simulink library "Steer_Rack"  (R2025a)
settings: Solver=VariableStepAuto  StartTime=0.0  StopTime=10.0  RelTol=1e-3
undefined symbols (not defined in the file): Vehicle
libraries: Steer_Rack_None x1, Steer_Rack_Only x1, Steer_Rack_RackDrivenShafts x1, Steer_Rack_RackStaticShafts x1, Steer_Rack_Wheel x1, Steer_Rack_WheelByWire x1, Steer_Rack_Wheel_Indep x1, Steer_Rack_WheelVarRatio x1, Steer_Rack_WheelDrivenRack x1, Steer_Rack_WheelDrivenRack1UJoint x1, Vehicle_Inputs x1
Description:
  | Component of Simscape Vehicle Templates Library
  | 
  | Copyright 2018-2026 The MathWorks, Inc.
settings Model: Creator=smiller  LastModifiedBy=smiller
settings SolverCC: AlgebraicLoopSolver=TrustRegion
settings DataIOCC: ReturnWorkspaceOutputs=off
settings OptimizationCC: ReuseModelBlockBuffer=off
settings DebuggingCC: UnconnectedInputMsg=warning  UnconnectedOutputMsg=warning  UnconnectedLineMsg=warning  ArithmeticOperatorsInVariantConditions=warning
settings ModelReferenceCC: EnableRefExpFcnMdlSchedulingChecks=on
settings SFSimCC: CustomCodeUndefinedFunction=UseInterfaceOnly
settings RTWCC: GPUComputeCapability=3.5  DLArmComputeVersion=19.05

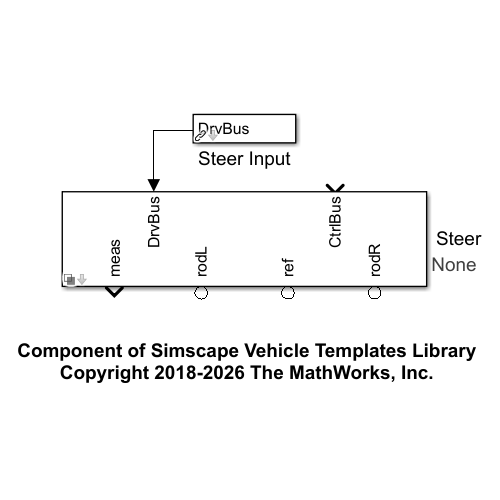
[thumbnail: Simulink's stored preview of the top-level diagram]
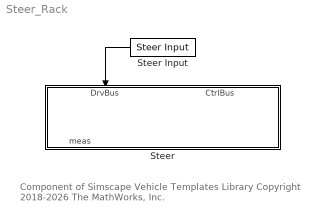
== system Steer_Rack ==
  note: Component of Simscape Vehicle Templates Library
      | Copyright 2018-2026 The MathWorks, Inc.
  Steer : Subsystem  Variant=on  VariantControlMode=label  VariantControl=Steer  LabelModeActiveChoice=None  mask(Steering System with Rack){Steer=Vehicle.Chassis.SuspF.Steer, VariantLabel=Vehicle.Chassis.SuspF.Steer.class.Value}
      mask prompts: Steer "Steer Parameters"; VariantLabel "Variant Label"
      mask help: Models steering system that involves a rack. Optionally include steering wheel. Connection between steering wheel and rack can be mechanical, specified by a lookup table, or a control system as in steer-by-wire. Option is chosen by string provided in Variant Label. The parameters for the selected option are contained in Steer data structure.
      mask init:
      | curblk = gcb;
      | 
      | % Set variant for this block 
      | set_param(curblk,'LabelModeActiveChoice',VariantLabel);
      settings: AttributesFormatString=%<ActiveVariant>
      mask Display: disp(' ');
  Steer Input : Vehicle_Inputs/DrvBus/Steer Input  popup_steer_input=Sequence
  wires:
  Steer Input/1 -> Steer/1(DrvBus)

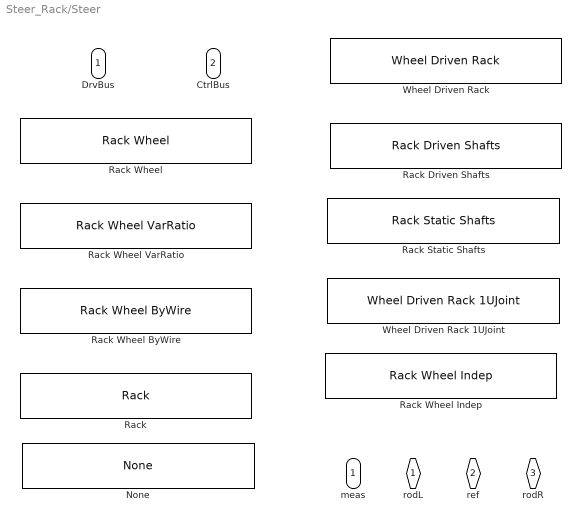
== system Steer_Rack/Steer ==
  DrvBus : Inport
  CtrlBus : Inport  Port=2
  None : Steer_Rack_None/None  SystemSampleTime=-1  VariantControl=None  VariantActivationTime=update diagram  EmptyChoice=off  PassThrough=off  PassThroughVariantControl=(default)  EmptyChoiceVariantControl=(default)  AllowFlexibleInterface=on  Latency=0  AutoFrameSizeCalculation=off
  Rack : Steer_Rack_Only/Rack  Tag=PublishSubsystem  VariantControl=Rack  hp_mt_rack=Steer.Rack.sMount.Value  hp_out_rack=Steer.Rack.sOutboard.Value  rack_mass=Steer.Rack.m.Value  whl2rack_whlangle=Steer.Ratio_Table.aWheel.Value  whl2rack_rackdisp=Steer.Ratio_Table.xRack.Value  whl2rack_filter=1/Steer.Rack.fActuatorCutoff.Value  clr_rack=Visual.SteeringRack.clr  opc_rack=Visual.part.opc  radius_rack=Visual.SteeringRack.rad  clr_connhp=Visual.hp.clr  opc_connhp=Visual.hp.opc  size_connhp=Visual.hp.rad
  Rack Driven Shafts : Steer_Rack_RackDrivenShafts/Rack Driven Shafts  Tag=PublishSubsystem  VariantControl=RackDrivenShafts  hp_wheel=Steer.Wheel.sMount.Value  wheel_axis_incl=Steer.Wheel.aAxis.Value  hp_mt_rack=Steer.Rack.sMount.Value  hp_out_rack=Steer.Rack.sOutboard.Value  hp_pinion=Steer.Pinion.sMount.Value  Wheel=Steer.Wheel  len_sha_u=Steer.Shaft_Upper.xLength.Value  sha_u_mass=Steer.Shaft_Upper.m.Value  sha_i_mass=Steer.Shaft_Intermediate.m.Value  len_sha_l=Steer.Shaft_Lower.xLength.Value  sha_l_mass=Steer.Shaft_Lower.m.Value  rad_pinion=Steer.Pinion.xRad.Value  pinion_mass=Steer.Pinion.m.Value  rack_mass=Steer.Rack.m.Value  whl2rack_whlangle=Steer.Ratio_Table.aWheel.Value  whl2rack_rackdisp=Steer.Ratio_Table.xRack.Value  steer_filter=1/Steer.Rack.fActuatorCutoff.Value  clr_rack=Visual.SteeringRack.clr  opc_rack=Visual.part.opc  radius_rack=Visual.SteeringRack.rad  clr_shaft=Visual.SteeringShafts.clr  opc_shaft=Visual.part.opc  size_shaft=Visual.SteeringShafts.rad  clr_pinion=Visual.SteeringPinion.clr  opc_pinion=Visual.part.opc  len_pinion=Visual.SteeringPinion.len  clr_connhp=Visual.hp.clr  opc_connhp=Visual.hp.opc  size_connhp=Visual.hp.rad  clr_wheel=Visual.SteeringWheel.clr  opc_wheel=Visual.part.opc  DriverHuman=Steer.DriverHuman
  Rack Static Shafts : Steer_Rack_RackStaticShafts/Rack Static Shafts  Tag=PublishSubsystem  VariantControl=RackStaticShafts  hp_wheel=Steer.Wheel.sMount.Value  wheel_axis_incl=Steer.Wheel.aAxis.Value  hp_mt_rack=Steer.Rack.sMount.Value  hp_out_rack=Steer.Rack.sOutboard.Value  hp_pinion=Steer.Pinion.sMount.Value  Wheel=Steer.Wheel  len_sha_u=Steer.Shaft_Upper.xLength.Value  sha_u_mass=Steer.Shaft_Upper.m.Value  sha_i_mass=Steer.Shaft_Intermediate.m.Value  len_sha_l=Steer.Shaft_Lower.xLength.Value  sha_l_mass=Steer.Shaft_Lower.m.Value  rad_pinion=Steer.Pinion.xRad.Value  pinion_mass=Steer.Pinion.m.Value  rack_mass=Steer.Rack.m.Value  whl2rack_whlangle=Steer.Ratio_Table.aWheel.Value  whl2rack_rackdisp=Steer.Ratio_Table.xRack.Value  steer_filter=1/Steer.Rack.fActuatorCutoff.Value  clr_rack=Visual.SteeringRack.clr  opc_rack=Visual.part.opc  radius_rack=Visual.SteeringRack.rad  clr_solid=Visual.SteeringShafts.clr  opc_solid=Visual.part.opc  rad_solid=Visual.SteeringShafts.rad  clr_pinion=Visual.SteeringPinion.clr  opc_pinion=Visual.part.opc  len_pinion=Visual.SteeringPinion.len  clr_connhp=Visual.hp.clr  opc_connhp=Visual.hp.opc  size_connhp=Visual.hp.rad  clr_wheel=Visual.SteeringWheel.clr  opc_wheel=Visual.part.opc  DriverHuman=Steer.DriverHuman
  Rack Wheel : Steer_Rack_Wheel/Rack Wheel  Tag=PublishSubsystem  VariantControl=RackWheel  hp_wheel=Steer.Wheel.sMount.Value  wheel_axis_incl=Steer.Wheel.aAxis.Value  hp_mt_rack=Steer.Rack.sMount.Value  hp_out_rack=Steer.Rack.sOutboard.Value  Wheel=Steer.Wheel  rack_mass=Steer.Rack.m.Value  whl2rack_whlangle=Steer.Ratio_Table.aWheel.Value  whl2rack_rackdisp=Steer.Ratio_Table.xRack.Value  whl2rack_filter=1/Steer.Rack.fActuatorCutoff.Value  clr_rack=Visual.SteeringRack.clr  opc_rack=Visual.part.opc  radius_rack=Visual.SteeringRack.rad  clr_connhp=Visual.hp.clr  opc_connhp=Visual.hp.opc  size_connhp=Visual.hp.rad  clr_wheel=Visual.SteeringWheel.clr  opc_wheel=Visual.part.opc  DriverHuman=Steer.DriverHuman
  Rack Wheel ByWire : Steer_Rack_WheelByWire/Rack Wheel ByWire  Tag=PublishSubsystem  VariantControl=RackWheelByWire  hp_wheel=Steer.Wheel.sMount.Value  wheel_axis_incl=Steer.Wheel.aAxis.Value  hp_mt_rack=Steer.Rack.sMount.Value  hp_out_rack=Steer.Rack.sOutboard.Value  Wheel=Steer.Wheel  rack_mass=Steer.Rack.m.Value  whl2rack_filter=1/Steer.Rack.fActuatorCutoff.Value  clr_rack=Visual.SteeringRack.clr  opc_rack=Visual.part.opc  radius_rack=Visual.SteeringRack.rad  clr_connhp=Visual.hp.clr  opc_connhp=Visual.hp.opc  size_connhp=Visual.hp.rad  clr_wheel=Visual.SteeringWheel.clr  opc_wheel=Visual.part.opc  DriverHuman=Steer.DriverHuman  Kp_breakpoints=Steer.Control.KpTable.xRack.Value  Kp_values=Steer.Control.KpTable.Kp.Value  Ki=Steer.Control.Ki.Value  Kd=Steer.Control.Kd.Value  tFilt_xRack=1/Steer.Control.fRackxCutoff.Value  tFilt_deriv=1/Steer.Control.fErrDerCutoff.Value  nTrqSteer=Steer.Control.nSteerTrq.Value  vDC=Steer.vMotor.Value  mSteer_trq=Steer.MotorSteer.TorqueSpd.trq.Value  mSteer_spd=Steer.MotorSteer.TorqueSpd.w.Value  mSteer_tc=1/Steer.MotorSteer.fActuatorCutoff.Value  mSteer_J=Steer.MotorSteer.J.Value  mSteer_d=Steer.MotorSteer.D.Value  mRack_trq=Steer.MotorRack.TorqueSpd.trq.Value  mRack_spd=Steer.MotorRack.TorqueSpd.w.Value  mRack_tc=1/Steer.MotorRack.fActuatorCutoff.Value  mRack_J=Steer.MotorRack.J.Value  mRack_d=Steer.MotorRack.D.Value  kRackCompliance=Steer.Rack.kCompliance.Value  DRackCompliance=Steer.Rack.DCompliance.Value  rPinion=Steer.Rack.xPinionRadius.Value  DRack=Steer.Rack.DHousing.Value
  Rack Wheel Indep : Steer_Rack_Wheel_Indep/Rack Wheel Indep  Tag=PublishSubsystem  VariantControl=RackWheelIndep  hp_wheel=Steer.Wheel.sMount.Value  wheel_axis_incl=Steer.Wheel.aAxis.Value  hp_mt_rack=Steer.Rack.sMount.Value  hp_out_rack=Steer.Rack.sOutboard.Value  Wheel=Steer.Wheel  rack_mass=Steer.Rack.m.Value  whl2rack_filter=1/Steer.Rack.fActuatorCutoff.Value  clr_rack=Visual.SteeringRack.clr  opc_rack=Visual.part.opc  radius_rack=Visual.SteeringRack.rad  clr_connhp=Visual.hp.clr  opc_connhp=Visual.hp.opc  size_connhp=Visual.hp.rad  clr_wheel=Visual.SteeringWheel.clr  opc_wheel=Visual.part.opc  DriverHuman=Steer.DriverHuman
  Rack Wheel VarRatio : Steer_Rack_WheelVarRatio/Rack Wheel VarRatio  Tag=PublishSubsystem  VariantControl=RackWheelVarRatio  hp_wheel=Steer.Wheel.sMount.Value  wheel_axis_incl=Steer.Wheel.aAxis.Value  hp_mt_rack=Steer.Rack.sMount.Value  hp_out_rack=Steer.Rack.sOutboard.Value  Wheel=Steer.Wheel  rack_mass=Steer.Rack.m.Value  whl2rack_filter=1/Steer.Rack.fActuatorCutoff.Value  clr_rack=Visual.SteeringRack.clr  opc_rack=Visual.part.opc  radius_rack=Visual.SteeringRack.rad  clr_connhp=Visual.hp.clr  opc_connhp=Visual.hp.opc  size_connhp=Visual.hp.rad  clr_wheel=Visual.SteeringWheel.clr  opc_wheel=Visual.part.opc  DriverHuman=Steer.DriverHuman  nTrqSteer=Steer.Control.nSteerTrq.Value  tFilt_forceFeedback=1/Steer.Control.fForceCutoff.Value
  Wheel Driven Rack : Steer_Rack_WheelDrivenRack/Wheel Driven Rack  Tag=PublishSubsystem  VariantControl=WheelDrivenRack  hp_wheel=Steer.Wheel.sMount.Value  wheel_axis_incl=Steer.Wheel.aAxis.Value  hp_mt_rack=Steer.Rack.sMount.Value  hp_out_rack=Steer.Rack.sOutboard.Value  hp_pinion=Steer.Pinion.sMount.Value  Wheel=Steer.Wheel  len_sha_u=Steer.Shaft_Upper.xLength.Value  sha_u_mass=Steer.Shaft_Upper.m.Value  sha_i_mass=Steer.Shaft_Intermediate.m.Value  len_sha_l=Steer.Shaft_Lower.xLength.Value  sha_l_mass=Steer.Shaft_Lower.m.Value  rad_pinion=Steer.Pinion.xRad.Value  pinion_mass=Steer.Pinion.m.Value  rack_mass=Steer.Rack.m.Value  whl2steer_filter=1/Steer.Rack.fActuatorCutoff.Value  clr_rack=Visual.SteeringRack.clr  opc_rack=Visual.part.opc  radius_rack=Visual.SteeringRack.rad  clr_shaft=Visual.SteeringShafts.clr  opc_shaft=Visual.part.opc  size_shaft=Visual.SteeringShafts.rad  clr_pinion=Visual.SteeringPinion.clr  opc_pinion=Visual.part.opc  len_pinion=Visual.SteeringPinion.len  clr_connhp=Visual.hp.clr  opc_connhp=Visual.hp.opc  size_connhp=Visual.hp.rad  clr_wheel=Visual.SteeringWheel.clr  opc_wheel=Visual.part.opc  DriverHuman=Steer.DriverHuman
  Wheel Driven Rack 1UJoint : Steer_Rack_WheelDrivenRack1UJoint/Wheel Driven Rack 1UJoint  Tag=PublishSubsystem  VariantControl=WheelDrivenRack1UJoint  hp_wheel=Steer.Wheel.sMount.Value  wheel_axis_incl=Steer.Wheel.aAxis.Value  hp_mt_rack=Steer.Rack.sMount.Value  hp_out_rack=Steer.Rack.sOutboard.Value  hp_pinion=Steer.Pinion.sMount.Value  Wheel=Steer.Wheel  len_sha_u=Steer.Shaft_Upper.xLength.Value  sha_u_mass=Steer.Shaft_Upper.m.Value  sha_l_mass=Steer.Shaft_Lower.m.Value  rad_pinion=Steer.Pinion.xRad.Value  pinion_mass=Steer.Pinion.m.Value  rack_mass=Steer.Rack.m.Value  whl2steer_filter=1/Steer.Rack.fActuatorCutoff.Value  clr_rack=Visual.SteeringRack.clr  opc_rack=Visual.part.opc  radius_rack=Visual.SteeringRack.rad  clr_shaft=Visual.SteeringShafts.clr  opc_shaft=Visual.part.opc  size_shaft=Visual.SteeringShafts.rad  clr_pinion=Visual.SteeringPinion.clr  opc_pinion=Visual.part.opc  len_pinion=Visual.SteeringPinion.len  clr_connhp=Visual.hp.clr  opc_connhp=Visual.hp.opc  size_connhp=Visual.hp.rad  clr_wheel=Visual.SteeringWheel.clr  opc_wheel=Visual.part.opc  DriverHuman=Steer.DriverHuman
  " rodL" : PMIOPort  Side=Right
  " ref" : PMIOPort  Port=2  Side=Right
  " rodR" : PMIOPort  Port=3  Side=Right
  " meas" : Outport  VectorParamsAs1DForOutWhenUnconnected=off
